simulink model "r2_b8a4x1kf"  (R2012b)
settings: Solver=VariableStepDiscrete  SolverMode=SingleTasking  StartTime=0.0  StopTime=1  RelTol=1e-3
undefined symbols (not defined in the file): fft_stages, n_bits_ants, n_bits_xengs
libraries: xbsIndex_r4 x22142, casper_library_misc x166, xbsReplacements_r4 x24, casper_library_delays x8, xps_library x5, casper_library_communications x4
(part 6 of 178)

== system r2_b8a4x1kf/bf1_ip ==
  io_delay : xbsIndex_r4/Delay  rst=off  infoeditControl=Selection of Reset will increase slice count due to use of real FFs and instead of SRLs  en=off  latency=0  dbl_ovrd=off  reg_retiming=on  block_type=delay
  r2_b8a4x1kf_new_bf1_ip_user_data_out : xbsIndex_r4/Gateway In  gui_display_data_type=Fixed-point  arith_type=Unsigned  n_bits=32  bin_pt=0  preci_type=Single  exp_width=8  frac_width=24  quantization="Round  (unbiased: +/- Inf)"  overflow=Saturate  period=1  dbl_ovrd=off  timing_constraint=None  locs_specified=off  LOCs={}  UseAsADC=off  ADCChannel='1'  inherit_from_input=off  hdl_port=on  block_type=gatewayin
  reint1 : xbsIndex_r4/Reinterpret  force_arith_type=on  arith_type=Unsigned  force_bin_pt=on  bin_pt=0  block_type=reinterpret
  sim_1 : Constant  Value=0
  slice_ip : xbsIndex_r4/Slice  nbits=32  boolean_output=off  mode=Lower Bit Location + Width  bit1=0  base1=MSB of Input  bit0=0  base0=LSB of Input  dbl_ovrd=off  block_type=slice
  in_ip : Outport
  wires:
  r2_b8a4x1kf_new_bf1_ip_user_data_out/1 -> io_delay/1
  sim_1/1 -> r2_b8a4x1kf_new_bf1_ip_user_data_out/1
  io_delay/1 -> slice_ip/1
  slice_ip/1 -> reint1/1
  reint1/1 -> in_ip/1

== system r2_b8a4x1kf/bf1_num_parts ==
  io_delay : xbsIndex_r4/Delay  rst=off  infoeditControl=Selection of Reset will increase slice count due to use of real FFs and instead of SRLs  en=off  latency=0  dbl_ovrd=off  reg_retiming=on  block_type=delay
  r2_b8a4x1kf_new_bf1_num_parts_user_data_out : xbsIndex_r4/Gateway In  gui_display_data_type=Fixed-point  arith_type=Unsigned  n_bits=32  bin_pt=0  preci_type=Single  exp_width=8  frac_width=24  quantization="Round  (unbiased: +/- Inf)"  overflow=Saturate  period=1  dbl_ovrd=off  timing_constraint=None  locs_specified=off  LOCs={}  UseAsADC=off  ADCChannel='1'  inherit_from_input=off  hdl_port=on  block_type=gatewayin
  reint1 : xbsIndex_r4/Reinterpret  force_arith_type=on  arith_type=Unsigned  force_bin_pt=on  bin_pt=0  block_type=reinterpret
  sim_1 : Constant  Value=0
  slice_n_partitions : xbsIndex_r4/Slice  nbits=6  boolean_output=off  mode=Lower Bit Location + Width  bit1=0  base1=MSB of Input  bit0=0  base0=LSB of Input  dbl_ovrd=off  block_type=slice
  in_n_partitions : Outport
  wires:
  r2_b8a4x1kf_new_bf1_num_parts_user_data_out/1 -> io_delay/1
  sim_1/1 -> r2_b8a4x1kf_new_bf1_num_parts_user_data_out/1
  io_delay/1 -> slice_n_partitions/1
  slice_n_partitions/1 -> reint1/1
  reint1/1 -> in_n_partitions/1

== system r2_b8a4x1kf/bf1_of_count ==
  out_count0 : Inport
  out_count1 : Inport  Port=2
  out_count2 : Inport  Port=3
  out_count3 : Inport  Port=4
  assert_count{0..3} (4 alike) : xbsIndex_r4/Assert  assert_type=on  type_source=Explicitly  gui_display_data_type=Fixed-point  arith_type=Unsigned  n_bits=8  bin_pt=0  preci_type=Single  exp_width=8  frac_width=24  assert_rate=off  rate_source=Explicitly  period=1  output_port=on  block_type=assert
  cast_gw : xbsIndex_r4/Convert  gui_display_data_type=Fixed-point  arith_type=Unsigned  n_bits=32  bin_pt=0  float_type=Single  exp_bits=8  fraction_bits=24  quantization=Truncate  overflow=Wrap  en=off  latency=0  dbl_ovrd=off  pipeline=off  block_type=convert
  concatenate : xbsIndex_r4/Concat  num_inputs=4  dbl_ovrd=off  block_type=concat
  io_delay : xbsIndex_r4/Delay  rst=off  infoeditControl=Selection of Reset will increase slice count due to use of real FFs and instead of SRLs  en=off  latency=0  dbl_ovrd=off  reg_retiming=on  block_type=delay
  r2_b8a4x1kf_new_bf1_of_count_user_data_in : xbsIndex_r4/Gateway Out  inherit_from_input=off  hdl_port=on  timing_constraint=None  locs_specified=off  LOCs={}  UseAsDAC=off  DACChannel='1'  block_type=gatewayout
  reint{1..4} (4 alike) : xbsIndex_r4/Reinterpret  force_arith_type=on  arith_type=Unsigned  force_bin_pt=on  bin_pt=0  block_type=reinterpret
  sim_out : Terminator
  wires:
  concatenate/1 -> io_delay/1
  io_delay/1 -> cast_gw/1
  cast_gw/1 -> r2_b8a4x1kf_new_bf1_of_count_user_data_in/1
  r2_b8a4x1kf_new_bf1_of_count_user_data_in/1 -> sim_out/1
  out_count0/1 -> assert_count0/1
  assert_count0/1 -> reint1/1
  reint1/1 -> concatenate/1
  out_count1/1 -> assert_count1/1
  assert_count1/1 -> reint2/1
  reint2/1 -> concatenate/2
  out_count2/1 -> assert_count2/1
  assert_count2/1 -> reint3/1
  reint3/1 -> concatenate/3
  out_count3/1 -> assert_count3/1
  assert_count3/1 -> reint4/1
  reint4/1 -> concatenate/4

== system r2_b8a4x1kf/bf1_out_count ==
  out_count0 : Inport
  out_count1 : Inport  Port=2
  out_count2 : Inport  Port=3
  out_count3 : Inport  Port=4
  assert_count{0..3} (4 alike) : xbsIndex_r4/Assert  assert_type=on  type_source=Explicitly  gui_display_data_type=Fixed-point  arith_type=Unsigned  n_bits=8  bin_pt=0  preci_type=Single  exp_width=8  frac_width=24  assert_rate=off  rate_source=Explicitly  period=1  output_port=on  block_type=assert
  cast_gw : xbsIndex_r4/Convert  gui_display_data_type=Fixed-point  arith_type=Unsigned  n_bits=32  bin_pt=0  float_type=Single  exp_bits=8  fraction_bits=24  quantization=Truncate  overflow=Wrap  en=off  latency=0  dbl_ovrd=off  pipeline=off  block_type=convert
  concatenate : xbsIndex_r4/Concat  num_inputs=4  dbl_ovrd=off  block_type=concat
  io_delay : xbsIndex_r4/Delay  rst=off  infoeditControl=Selection of Reset will increase slice count due to use of real FFs and instead of SRLs  en=off  latency=0  dbl_ovrd=off  reg_retiming=on  block_type=delay
  r2_b8a4x1kf_new_bf1_out_count_user_data_in : xbsIndex_r4/Gateway Out  inherit_from_input=off  hdl_port=on  timing_constraint=None  locs_specified=off  LOCs={}  UseAsDAC=off  DACChannel='1'  block_type=gatewayout
  reint{1..4} (4 alike) : xbsIndex_r4/Reinterpret  force_arith_type=on  arith_type=Unsigned  force_bin_pt=on  bin_pt=0  block_type=reinterpret
  sim_out : Terminator
  wires:
  concatenate/1 -> io_delay/1
  io_delay/1 -> cast_gw/1
  cast_gw/1 -> r2_b8a4x1kf_new_bf1_out_count_user_data_in/1
  r2_b8a4x1kf_new_bf1_out_count_user_data_in/1 -> sim_out/1
  out_count0/1 -> assert_count0/1
  assert_count0/1 -> reint1/1
  reint1/1 -> concatenate/1
  out_count1/1 -> assert_count1/1
  assert_count1/1 -> reint2/1
  reint2/1 -> concatenate/2
  out_count2/1 -> assert_count2/1
  assert_count2/1 -> reint3/1
  reint3/1 -> concatenate/3
  out_count3/1 -> assert_count3/1
  assert_count3/1 -> reint4/1
  reint4/1 -> concatenate/4

== system r2_b8a4x1kf/bf1_partitions ==
  convert1_{1..4} (4 alike) : DataTypeConversion  OutDataTypeStr=fixdt('ufix5_En0')  LockScale=on
  convert2_{1..4} (4 alike) : DataTypeConversion  OutDataTypeStr=fixdt('ufix5_En0')  ConvertRealWorld=Stored Integer (SI)  LockScale=on
  gain_1 : Gain  Gain=32768
  gain_2 : Gain  Gain=1024
  gain_3 : Gain  Gain=32
  gain_4 : Gain
  io_delay : xbsIndex_r4/Delay  rst=off  infoeditControl=Selection of Reset will increase slice count due to use of real FFs and instead of SRLs  en=off  latency=0  dbl_ovrd=off  reg_retiming=on  block_type=delay
  r2_b8a4x1kf_new_bf1_partitions_user_data_out : xbsIndex_r4/Gateway In  gui_display_data_type=Fixed-point  arith_type=Unsigned  n_bits=32  bin_pt=0  preci_type=Single  exp_width=8  frac_width=24  quantization="Round  (unbiased: +/- Inf)"  overflow=Saturate  period=1  dbl_ovrd=off  timing_constraint=None  locs_specified=off  LOCs={}  UseAsADC=off  ADCChannel='1'  inherit_from_input=off  hdl_port=on  block_type=gatewayin
  reint{1..4} (4 alike) : xbsIndex_r4/Reinterpret  force_arith_type=on  arith_type=Unsigned  force_bin_pt=on  bin_pt=0  block_type=reinterpret
  sim_{1..4} (4 alike) : Constant  Value=0
  sim_add : Sum  Inputs=++++  OutDataTypeStr=uint32
  slice_partition0_offset : xbsIndex_r4/Slice  nbits=5  boolean_output=off  mode=Lower Bit Location + Width  bit1=0  base1=MSB of Input  bit0=15  base0=LSB of Input  dbl_ovrd=off  block_type=slice
  slice_partition1_offset : xbsIndex_r4/Slice  nbits=5  boolean_output=off  mode=Lower Bit Location + Width  bit1=0  base1=MSB of Input  bit0=10  base0=LSB of Input  dbl_ovrd=off  block_type=slice
  slice_partition2_offset : xbsIndex_r4/Slice  nbits=5  boolean_output=off  mode=Lower Bit Location + Width  bit1=0  base1=MSB of Input  bit0=5  base0=LSB of Input  dbl_ovrd=off  block_type=slice
  slice_partition3_offset : xbsIndex_r4/Slice  nbits=5  boolean_output=off  mode=Lower Bit Location + Width  bit1=0  base1=MSB of Input  bit0=0  base0=LSB of Input  dbl_ovrd=off  block_type=slice
  in_partition0_offset : Outport
  in_partition1_offset : Outport  Port=2
  in_partition2_offset : Outport  Port=3
  in_partition3_offset : Outport  Port=4
  wires:
  r2_b8a4x1kf_new_bf1_partitions_user_data_out/1 -> io_delay/1
  sim_add/1 -> r2_b8a4x1kf_new_bf1_partitions_user_data_out/1
  sim_1/1 -> convert1_1/1
  convert1_1/1 -> convert2_1/1
  convert2_1/1 -> gain_1/1
  gain_1/1 -> sim_add/1
  io_delay/1 -> slice_partition0_offset/1, slice_partition1_offset/1, slice_partition2_offset/1, slice_partition3_offset/1
  slice_partition0_offset/1 -> reint1/1
  reint1/1 -> in_partition0_offset/1
  sim_2/1 -> convert1_2/1
  convert1_2/1 -> convert2_2/1
  convert2_2/1 -> gain_2/1
  gain_2/1 -> sim_add/2
  slice_partition1_offset/1 -> reint2/1
  reint2/1 -> in_partition1_offset/1
  sim_3/1 -> convert1_3/1
  convert1_3/1 -> convert2_3/1
  convert2_3/1 -> gain_3/1
  gain_3/1 -> sim_add/3
  slice_partition2_offset/1 -> reint3/1
  reint3/1 -> in_partition2_offset/1
  sim_4/1 -> convert1_4/1
  convert1_4/1 -> convert2_4/1
  convert2_4/1 -> gain_4/1
  gain_4/1 -> sim_add/4
  slice_partition3_offset/1 -> reint4/1
  reint4/1 -> in_partition3_offset/1

== system r2_b8a4x1kf/bf_config ==
  convert1_1 : DataTypeConversion  OutDataTypeStr=fixdt('ufix8_En0')  LockScale=on
  convert1_2 : DataTypeConversion  OutDataTypeStr=fixdt('ufix16_En0')  LockScale=on
  convert1_3 : DataTypeConversion  OutDataTypeStr=fixdt('ufix1_En0')  LockScale=on
  convert1_4 : DataTypeConversion  OutDataTypeStr=fixdt('ufix1_En0')  LockScale=on
  convert1_5 : DataTypeConversion  OutDataTypeStr=fixdt('ufix1_En0')  LockScale=on
  convert2_1 : DataTypeConversion  OutDataTypeStr=fixdt('ufix8_En0')  ConvertRealWorld=Stored Integer (SI)  LockScale=on
  convert2_2 : DataTypeConversion  OutDataTypeStr=fixdt('ufix16_En0')  ConvertRealWorld=Stored Integer (SI)  LockScale=on
  convert2_3 : DataTypeConversion  OutDataTypeStr=fixdt('ufix1_En0')  ConvertRealWorld=Stored Integer (SI)  LockScale=on
  convert2_4 : DataTypeConversion  OutDataTypeStr=fixdt('ufix1_En0')  ConvertRealWorld=Stored Integer (SI)  LockScale=on
  convert2_5 : DataTypeConversion  OutDataTypeStr=fixdt('ufix1_En0')  ConvertRealWorld=Stored Integer (SI)  LockScale=on
  gain_1 : Gain  Gain=524288
  gain_2 : Gain  Gain=8
  gain_3 : Gain  Gain=4
  gain_4 : Gain  Gain=2
  gain_5 : Gain
  io_delay : xbsIndex_r4/Delay  rst=off  infoeditControl=Selection of Reset will increase slice count due to use of real FFs and instead of SRLs  en=off  latency=0  dbl_ovrd=off  reg_retiming=on  block_type=delay
  r2_b8a4x1kf_new_bf_config_user_data_out : xbsIndex_r4/Gateway In  gui_display_data_type=Fixed-point  arith_type=Unsigned  n_bits=32  bin_pt=0  preci_type=Single  exp_width=8  frac_width=24  quantization="Round  (unbiased: +/- Inf)"  overflow=Saturate  period=1  dbl_ovrd=off  timing_constraint=None  locs_specified=off  LOCs={}  UseAsADC=off  ADCChannel='1'  inherit_from_input=off  hdl_port=on  block_type=gatewayin
  reint1 : xbsIndex_r4/Reinterpret  force_arith_type=on  arith_type=Unsigned  force_bin_pt=on  bin_pt=0  block_type=reinterpret
  reint2 : xbsIndex_r4/Reinterpret  force_arith_type=on  arith_type=Unsigned  force_bin_pt=on  bin_pt=0  block_type=reinterpret
  sim_{1..5} (5 alike) : Constant  Value=0
  sim_add : Sum  Inputs=+++++  OutDataTypeStr=uint32
  slice_data_id : xbsIndex_r4/Slice  nbits=8  boolean_output=off  mode=Lower Bit Location + Width  bit1=0  base1=MSB of Input  bit0=19  base0=LSB of Input  dbl_ovrd=off  block_type=slice
  slice_snap_arm : xbsIndex_r4/Slice  nbits=1  boolean_output=on  mode=Lower Bit Location + Width  bit1=0  base1=MSB of Input  bit0=1  base0=LSB of Input  dbl_ovrd=off  block_type=slice
  slice_snap_trig : xbsIndex_r4/Slice  nbits=1  boolean_output=on  mode=Lower Bit Location + Width  bit1=0  base1=MSB of Input  bit0=0  base0=LSB of Input  dbl_ovrd=off  block_type=slice
  slice_time_id : xbsIndex_r4/Slice  nbits=16  boolean_output=off  mode=Lower Bit Location + Width  bit1=0  base1=MSB of Input  bit0=3  base0=LSB of Input  dbl_ovrd=off  block_type=slice
  slice_tvg_sel : xbsIndex_r4/Slice  nbits=1  boolean_output=on  mode=Lower Bit Location + Width  bit1=0  base1=MSB of Input  bit0=2  base0=LSB of Input  dbl_ovrd=off  block_type=slice
  in_data_id : Outport
  in_time_id : Outport  Port=2
  in_tvg_sel : Outport  Port=3
  in_snap_arm : Outport  Port=4
  in_snap_trig : Outport  Port=5
  wires:
  r2_b8a4x1kf_new_bf_config_user_data_out/1 -> io_delay/1
  sim_add/1 -> r2_b8a4x1kf_new_bf_config_user_data_out/1
  sim_1/1 -> convert1_1/1
  convert1_1/1 -> convert2_1/1
  convert2_1/1 -> gain_1/1
  gain_1/1 -> sim_add/1
  io_delay/1 -> slice_data_id/1, slice_time_id/1, slice_tvg_sel/1, slice_snap_arm/1, slice_snap_trig/1
  slice_data_id/1 -> reint1/1
  reint1/1 -> in_data_id/1
  sim_2/1 -> convert1_2/1
  convert1_2/1 -> convert2_2/1
  convert2_2/1 -> gain_2/1
  gain_2/1 -> sim_add/2
  slice_time_id/1 -> reint2/1
  reint2/1 -> in_time_id/1
  sim_3/1 -> convert1_3/1
  convert1_3/1 -> convert2_3/1
  convert2_3/1 -> gain_3/1
  gain_3/1 -> sim_add/3
  slice_tvg_sel/1 -> in_tvg_sel/1
  sim_4/1 -> convert1_4/1
  convert1_4/1 -> convert2_4/1
  convert2_4/1 -> gain_4/1
  gain_4/1 -> sim_add/4
  slice_snap_arm/1 -> in_snap_arm/1
  sim_5/1 -> convert1_5/1
  convert1_5/1 -> convert2_5/1
  convert2_5/1 -> gain_5/1
  gain_5/1 -> sim_add/5
  slice_snap_trig/1 -> in_snap_trig/1

== system r2_b8a4x1kf/bf_control ==
  convert1_1 : DataTypeConversion  OutDataTypeStr=fixdt('ufix2_En0')  LockScale=on
  convert1_2 : DataTypeConversion  OutDataTypeStr=fixdt('ufix1_En0')  LockScale=on
  convert1_3 : DataTypeConversion  OutDataTypeStr=fixdt('ufix3_En0')  LockScale=on
  convert2_1 : DataTypeConversion  OutDataTypeStr=fixdt('ufix2_En0')  ConvertRealWorld=Stored Integer (SI)  LockScale=on
  convert2_2 : DataTypeConversion  OutDataTypeStr=fixdt('ufix1_En0')  ConvertRealWorld=Stored Integer (SI)  LockScale=on
  convert2_3 : DataTypeConversion  OutDataTypeStr=fixdt('ufix3_En0')  ConvertRealWorld=Stored Integer (SI)  LockScale=on
  gain_1 : Gain  Gain=16
  gain_2 : Gain  Gain=8
  gain_3 : Gain
  io_delay : xbsIndex_r4/Delay  rst=off  infoeditControl=Selection of Reset will increase slice count due to use of real FFs and instead of SRLs  en=off  latency=0  dbl_ovrd=off  reg_retiming=on  block_type=delay
  r2_b8a4x1kf_new_bf_control_user_data_out : xbsIndex_r4/Gateway In  gui_display_data_type=Fixed-point  arith_type=Unsigned  n_bits=32  bin_pt=0  preci_type=Single  exp_width=8  frac_width=24  quantization="Round  (unbiased: +/- Inf)"  overflow=Saturate  period=1  dbl_ovrd=off  timing_constraint=None  locs_specified=off  LOCs={}  UseAsADC=off  ADCChannel='1'  inherit_from_input=off  hdl_port=on  block_type=gatewayin
  reint1 : xbsIndex_r4/Reinterpret  force_arith_type=on  arith_type=Unsigned  force_bin_pt=on  bin_pt=0  block_type=reinterpret
  reint2 : xbsIndex_r4/Reinterpret  force_arith_type=on  arith_type=Unsigned  force_bin_pt=on  bin_pt=0  block_type=reinterpret
  reint3 : xbsIndex_r4/Reinterpret  force_arith_type=on  arith_type=Unsigned  force_bin_pt=on  bin_pt=0  block_type=reinterpret
  sim_1 : Constant  Value=0
  sim_2 : Constant  Value=0
  sim_3 : Constant  Value=0
  sim_add : Sum  Inputs=+++  OutDataTypeStr=uint32
  slice_antenna : xbsIndex_r4/Slice  nbits=3  boolean_output=off  mode=Lower Bit Location + Width  bit1=0  base1=MSB of Input  bit0=0  base0=LSB of Input  dbl_ovrd=off  block_type=slice
  slice_beng : xbsIndex_r4/Slice  nbits=2  boolean_output=off  mode=Lower Bit Location + Width  bit1=0  base1=MSB of Input  bit0=4  base0=LSB of Input  dbl_ovrd=off  block_type=slice
  slice_stream : xbsIndex_r4/Slice  nbits=1  boolean_output=off  mode=Lower Bit Location + Width  bit1=0  base1=MSB of Input  bit0=3  base0=LSB of Input  dbl_ovrd=off  block_type=slice
  in_beng : Outport
  in_stream : Outport  Port=2
  in_antenna : Outport  Port=3
  wires:
  r2_b8a4x1kf_new_bf_control_user_data_out/1 -> io_delay/1
  sim_add/1 -> r2_b8a4x1kf_new_bf_control_user_data_out/1
  sim_1/1 -> convert1_1/1
  convert1_1/1 -> convert2_1/1
  convert2_1/1 -> gain_1/1
  gain_1/1 -> sim_add/1
  io_delay/1 -> slice_beng/1, slice_stream/1, slice_antenna/1
  slice_beng/1 -> reint1/1
  reint1/1 -> in_beng/1
  sim_2/1 -> convert1_2/1
  convert1_2/1 -> convert2_2/1
  convert2_2/1 -> gain_2/1
  gain_2/1 -> sim_add/2
  slice_stream/1 -> reint2/1
  reint2/1 -> in_stream/1
  sim_3/1 -> convert1_3/1
  convert1_3/1 -> convert2_3/1
  convert2_3/1 -> gain_3/1
  gain_3/1 -> sim_add/3
  slice_antenna/1 -> reint3/1
  reint3/1 -> in_antenna/1

== system r2_b8a4x1kf/bf_valout_bw0 ==
  out_bw0 : Inport
  out_bw1 : Inport  Port=2
  assert_bw0 : xbsIndex_r4/Assert  assert_type=on  type_source=Explicitly  gui_display_data_type=Fixed-point  arith_type="Signed  (2's comp)"  n_bits=16  bin_pt=9  preci_type=Single  exp_width=8  frac_width=24  assert_rate=off  rate_source=Explicitly  period=1  output_port=on  block_type=assert
  assert_bw1 : xbsIndex_r4/Assert  assert_type=on  type_source=Explicitly  gui_display_data_type=Fixed-point  arith_type="Signed  (2's comp)"  n_bits=16  bin_pt=9  preci_type=Single  exp_width=8  frac_width=24  assert_rate=off  rate_source=Explicitly  period=1  output_port=on  block_type=assert
  cast_gw : xbsIndex_r4/Convert  gui_display_data_type=Fixed-point  arith_type=Unsigned  n_bits=32  bin_pt=0  float_type=Single  exp_bits=8  fraction_bits=24  quantization=Truncate  overflow=Wrap  en=off  latency=0  dbl_ovrd=off  pipeline=off  block_type=convert
  concatenate : xbsIndex_r4/Concat  num_inputs=2  dbl_ovrd=off  block_type=concat
  io_delay : xbsIndex_r4/Delay  rst=off  infoeditControl=Selection of Reset will increase slice count due to use of real FFs and instead of SRLs  en=off  latency=1  dbl_ovrd=off  reg_retiming=on  block_type=delay
  r2_b8a4x1kf_new_bf_valout_bw0_user_data_in : xbsIndex_r4/Gateway Out  inherit_from_input=off  hdl_port=on  timing_constraint=None  locs_specified=off  LOCs={}  UseAsDAC=off  DACChannel='1'  block_type=gatewayout
  reint1 : xbsIndex_r4/Reinterpret  force_arith_type=on  arith_type=Unsigned  force_bin_pt=on  bin_pt=0  block_type=reinterpret
  reint2 : xbsIndex_r4/Reinterpret  force_arith_type=on  arith_type=Unsigned  force_bin_pt=on  bin_pt=0  block_type=reinterpret
  sim_out : Terminator
  wires:
  concatenate/1 -> io_delay/1
  io_delay/1 -> cast_gw/1
  cast_gw/1 -> r2_b8a4x1kf_new_bf_valout_bw0_user_data_in/1
  r2_b8a4x1kf_new_bf_valout_bw0_user_data_in/1 -> sim_out/1
  out_bw0/1 -> assert_bw0/1
  assert_bw0/1 -> reint1/1
  reint1/1 -> concatenate/1
  out_bw1/1 -> assert_bw1/1
  assert_bw1/1 -> reint2/1
  reint2/1 -> concatenate/2

== system r2_b8a4x1kf/bf_valout_bw1 ==
  out_bw2 : Inport
  out_bw3 : Inport  Port=2
  assert_bw2 : xbsIndex_r4/Assert  assert_type=on  type_source=Explicitly  gui_display_data_type=Fixed-point  arith_type="Signed  (2's comp)"  n_bits=16  bin_pt=9  preci_type=Single  exp_width=8  frac_width=24  assert_rate=off  rate_source=Explicitly  period=1  output_port=on  block_type=assert
  assert_bw3 : xbsIndex_r4/Assert  assert_type=on  type_source=Explicitly  gui_display_data_type=Fixed-point  arith_type="Signed  (2's comp)"  n_bits=16  bin_pt=9  preci_type=Single  exp_width=8  frac_width=24  assert_rate=off  rate_source=Explicitly  period=1  output_port=on  block_type=assert
  cast_gw : xbsIndex_r4/Convert  gui_display_data_type=Fixed-point  arith_type=Unsigned  n_bits=32  bin_pt=0  float_type=Single  exp_bits=8  fraction_bits=24  quantization=Truncate  overflow=Wrap  en=off  latency=0  dbl_ovrd=off  pipeline=off  block_type=convert
  concatenate : xbsIndex_r4/Concat  num_inputs=2  dbl_ovrd=off  block_type=concat
  io_delay : xbsIndex_r4/Delay  rst=off  infoeditControl=Selection of Reset will increase slice count due to use of real FFs and instead of SRLs  en=off  latency=1  dbl_ovrd=off  reg_retiming=on  block_type=delay
  r2_b8a4x1kf_new_bf_valout_bw1_user_data_in : xbsIndex_r4/Gateway Out  inherit_from_input=off  hdl_port=on  timing_constraint=None  locs_specified=off  LOCs={}  UseAsDAC=off  DACChannel='1'  block_type=gatewayout
  reint1 : xbsIndex_r4/Reinterpret  force_arith_type=on  arith_type=Unsigned  force_bin_pt=on  bin_pt=0  block_type=reinterpret
  reint2 : xbsIndex_r4/Reinterpret  force_arith_type=on  arith_type=Unsigned  force_bin_pt=on  bin_pt=0  block_type=reinterpret
  sim_out : Terminator
  wires:
  concatenate/1 -> io_delay/1
  io_delay/1 -> cast_gw/1
  cast_gw/1 -> r2_b8a4x1kf_new_bf_valout_bw1_user_data_in/1
  r2_b8a4x1kf_new_bf_valout_bw1_user_data_in/1 -> sim_out/1
  out_bw2/1 -> assert_bw2/1
  assert_bw2/1 -> reint1/1
  reint1/1 -> concatenate/1
  out_bw3/1 -> assert_bw3/1
  assert_bw3/1 -> reint2/1
  reint2/1 -> concatenate/2

== system r2_b8a4x1kf/bf_valout_filt ==
  out_filt0 : Inport
  out_filt1 : Inport  Port=2
  out_filt2 : Inport  Port=3
  out_filt3 : Inport  Port=4
  assert_filt{0..3} (4 alike) : xbsIndex_r4/Assert  assert_type=on  type_source=Explicitly  gui_display_data_type=Fixed-point  arith_type=Unsigned  n_bits=1  bin_pt=0  preci_type=Single  exp_width=8  frac_width=24  assert_rate=off  rate_source=Explicitly  period=1  output_port=on  block_type=assert
  cast_gw : xbsIndex_r4/Convert  gui_display_data_type=Fixed-point  arith_type=Unsigned  n_bits=32  bin_pt=0  float_type=Single  exp_bits=8  fraction_bits=24  quantization=Truncate  overflow=Wrap  en=off  latency=0  dbl_ovrd=off  pipeline=off  block_type=convert
  concatenate : xbsIndex_r4/Concat  num_inputs=4  dbl_ovrd=off  block_type=concat
  io_delay : xbsIndex_r4/Delay  rst=off  infoeditControl=Selection of Reset will increase slice count due to use of real FFs and instead of SRLs  en=off  latency=1  dbl_ovrd=off  reg_retiming=on  block_type=delay
  r2_b8a4x1kf_new_bf_valout_filt_user_data_in : xbsIndex_r4/Gateway Out  inherit_from_input=off  hdl_port=on  timing_constraint=None  locs_specified=off  LOCs={}  UseAsDAC=off  DACChannel='1'  block_type=gatewayout
  reint{1..4} (4 alike) : xbsIndex_r4/Reinterpret  force_arith_type=on  arith_type=Unsigned  force_bin_pt=on  bin_pt=0  block_type=reinterpret
  sim_out : Terminator
  wires:
  concatenate/1 -> io_delay/1
  io_delay/1 -> cast_gw/1
  cast_gw/1 -> r2_b8a4x1kf_new_bf_valout_filt_user_data_in/1
  r2_b8a4x1kf_new_bf_valout_filt_user_data_in/1 -> sim_out/1
  out_filt0/1 -> assert_filt0/1
  assert_filt0/1 -> reint1/1
  reint1/1 -> concatenate/1
  out_filt1/1 -> assert_filt1/1
  assert_filt1/1 -> reint2/1
  reint2/1 -> concatenate/2
  out_filt2/1 -> assert_filt2/1
  assert_filt2/1 -> reint3/1
  reint3/1 -> concatenate/3
  out_filt3/1 -> assert_filt3/1
  assert_filt3/1 -> reint4/1
  reint4/1 -> concatenate/4

== system r2_b8a4x1kf/bf_valout_quant0 ==
  out_quant0 : Inport
  out_quant1 : Inport  Port=2
  assert_quant0 : xbsIndex_r4/Assert  assert_type=on  type_source=Explicitly  gui_display_data_type=Fixed-point  arith_type="Signed  (2's comp)"  n_bits=16  bin_pt=8  preci_type=Single  exp_width=8  frac_width=24  assert_rate=off  rate_source=Explicitly  period=1  output_port=on  block_type=assert
  assert_quant1 : xbsIndex_r4/Assert  assert_type=on  type_source=Explicitly  gui_display_data_type=Fixed-point  arith_type="Signed  (2's comp)"  n_bits=16  bin_pt=8  preci_type=Single  exp_width=8  frac_width=24  assert_rate=off  rate_source=Explicitly  period=1  output_port=on  block_type=assert
  cast_gw : xbsIndex_r4/Convert  gui_display_data_type=Fixed-point  arith_type=Unsigned  n_bits=32  bin_pt=0  float_type=Single  exp_bits=8  fraction_bits=24  quantization=Truncate  overflow=Wrap  en=off  latency=0  dbl_ovrd=off  pipeline=off  block_type=convert
  concatenate : xbsIndex_r4/Concat  num_inputs=2  dbl_ovrd=off  block_type=concat
  io_delay : xbsIndex_r4/Delay  rst=off  infoeditControl=Selection of Reset will increase slice count due to use of real FFs and instead of SRLs  en=off  latency=1  dbl_ovrd=off  reg_retiming=on  block_type=delay
  r2_b8a4x1kf_new_bf_valout_quant0_user_data_in : xbsIndex_r4/Gateway Out  inherit_from_input=off  hdl_port=on  timing_constraint=None  locs_specified=off  LOCs={}  UseAsDAC=off  DACChannel='1'  block_type=gatewayout
  reint1 : xbsIndex_r4/Reinterpret  force_arith_type=on  arith_type=Unsigned  force_bin_pt=on  bin_pt=0  block_type=reinterpret
  reint2 : xbsIndex_r4/Reinterpret  force_arith_type=on  arith_type=Unsigned  force_bin_pt=on  bin_pt=0  block_type=reinterpret
  sim_out : Terminator
  wires:
  concatenate/1 -> io_delay/1
  io_delay/1 -> cast_gw/1
  cast_gw/1 -> r2_b8a4x1kf_new_bf_valout_quant0_user_data_in/1
  r2_b8a4x1kf_new_bf_valout_quant0_user_data_in/1 -> sim_out/1
  out_quant0/1 -> assert_quant0/1
  assert_quant0/1 -> reint1/1
  reint1/1 -> concatenate/1
  out_quant1/1 -> assert_quant1/1
  assert_quant1/1 -> reint2/1
  reint2/1 -> concatenate/2

== system r2_b8a4x1kf/bf_valout_quant1 ==
  out_quant2 : Inport
  out_quant3 : Inport  Port=2
  assert_quant2 : xbsIndex_r4/Assert  assert_type=on  type_source=Explicitly  gui_display_data_type=Fixed-point  arith_type="Signed  (2's comp)"  n_bits=16  bin_pt=8  preci_type=Single  exp_width=8  frac_width=24  assert_rate=off  rate_source=Explicitly  period=1  output_port=on  block_type=assert
  assert_quant3 : xbsIndex_r4/Assert  assert_type=on  type_source=Explicitly  gui_display_data_type=Fixed-point  arith_type="Signed  (2's comp)"  n_bits=16  bin_pt=8  preci_type=Single  exp_width=8  frac_width=24  assert_rate=off  rate_source=Explicitly  period=1  output_port=on  block_type=assert
  cast_gw : xbsIndex_r4/Convert  gui_display_data_type=Fixed-point  arith_type=Unsigned  n_bits=32  bin_pt=0  float_type=Single  exp_bits=8  fraction_bits=24  quantization=Truncate  overflow=Wrap  en=off  latency=0  dbl_ovrd=off  pipeline=off  block_type=convert
  concatenate : xbsIndex_r4/Concat  num_inputs=2  dbl_ovrd=off  block_type=concat
  io_delay : xbsIndex_r4/Delay  rst=off  infoeditControl=Selection of Reset will increase slice count due to use of real FFs and instead of SRLs  en=off  latency=1  dbl_ovrd=off  reg_retiming=on  block_type=delay
  r2_b8a4x1kf_new_bf_valout_quant1_user_data_in : xbsIndex_r4/Gateway Out  inherit_from_input=off  hdl_port=on  timing_constraint=None  locs_specified=off  LOCs={}  UseAsDAC=off  DACChannel='1'  block_type=gatewayout
  reint1 : xbsIndex_r4/Reinterpret  force_arith_type=on  arith_type=Unsigned  force_bin_pt=on  bin_pt=0  block_type=reinterpret
  reint2 : xbsIndex_r4/Reinterpret  force_arith_type=on  arith_type=Unsigned  force_bin_pt=on  bin_pt=0  block_type=reinterpret
  sim_out : Terminator
  wires:
  concatenate/1 -> io_delay/1
  io_delay/1 -> cast_gw/1
  cast_gw/1 -> r2_b8a4x1kf_new_bf_valout_quant1_user_data_in/1
  r2_b8a4x1kf_new_bf_valout_quant1_user_data_in/1 -> sim_out/1
  out_quant2/1 -> assert_quant2/1
  assert_quant2/1 -> reint1/1
  reint1/1 -> concatenate/1
  out_quant3/1 -> assert_quant3/1
  assert_quant3/1 -> reint2/1
  reint2/1 -> concatenate/2

== system r2_b8a4x1kf/bf_value_ctrl ==
  convert1_{1..4} (4 alike) : DataTypeConversion  OutDataTypeStr=fixdt('ufix1_En0')  LockScale=on
  convert2_{1..4} (4 alike) : DataTypeConversion  OutDataTypeStr=fixdt('ufix1_En0')  ConvertRealWorld=Stored Integer (SI)  LockScale=on
  gain_1 : Gain  Gain=8
  gain_2 : Gain  Gain=4
  gain_3 : Gain  Gain=2
  gain_4 : Gain
  io_delay : xbsIndex_r4/Delay  rst=off  infoeditControl=Selection of Reset will increase slice count due to use of real FFs and instead of SRLs  en=off  latency=0  dbl_ovrd=off  reg_retiming=on  block_type=delay
  r2_b8a4x1kf_new_bf_value_ctrl_user_data_out : xbsIndex_r4/Gateway In  gui_display_data_type=Fixed-point  arith_type=Unsigned  n_bits=32  bin_pt=0  preci_type=Single  exp_width=8  frac_width=24  quantization="Round  (unbiased: +/- Inf)"  overflow=Saturate  period=1  dbl_ovrd=off  timing_constraint=None  locs_specified=off  LOCs={}  UseAsADC=off  ADCChannel='1'  inherit_from_input=off  hdl_port=on  block_type=gatewayin
  sim_{1..4} (4 alike) : Constant  Value=0
  sim_add : Sum  Inputs=++++  OutDataTypeStr=uint32
  slice_bw : xbsIndex_r4/Slice  nbits=1  boolean_output=on  mode=Lower Bit Location + Width  bit1=0  base1=MSB of Input  bit0=2  base0=LSB of Input  dbl_ovrd=off  block_type=slice
  slice_dupl : xbsIndex_r4/Slice  nbits=1  boolean_output=on  mode=Lower Bit Location + Width  bit1=0  base1=MSB of Input  bit0=3  base0=LSB of Input  dbl_ovrd=off  block_type=slice
  slice_filt : xbsIndex_r4/Slice  nbits=1  boolean_output=on  mode=Lower Bit Location + Width  bit1=0  base1=MSB of Input  bit0=0  base0=LSB of Input  dbl_ovrd=off  block_type=slice
  slice_quant : xbsIndex_r4/Slice  nbits=1  boolean_output=on  mode=Lower Bit Location + Width  bit1=0  base1=MSB of Input  bit0=1  base0=LSB of Input  dbl_ovrd=off  block_type=slice
  in_dupl : Outport
  in_bw : Outport  Port=2
  in_quant : Outport  Port=3
  in_filt : Outport  Port=4
  wires:
  r2_b8a4x1kf_new_bf_value_ctrl_user_data_out/1 -> io_delay/1
  sim_add/1 -> r2_b8a4x1kf_new_bf_value_ctrl_user_data_out/1
  sim_1/1 -> convert1_1/1
  convert1_1/1 -> convert2_1/1
  convert2_1/1 -> gain_1/1
  gain_1/1 -> sim_add/1
  io_delay/1 -> slice_dupl/1, slice_bw/1, slice_quant/1, slice_filt/1
  slice_dupl/1 -> in_dupl/1
  sim_2/1 -> convert1_2/1
  convert1_2/1 -> convert2_2/1
  convert2_2/1 -> gain_2/1
  gain_2/1 -> sim_add/2
  slice_bw/1 -> in_bw/1
  sim_3/1 -> convert1_3/1
  convert1_3/1 -> convert2_3/1
  convert2_3/1 -> gain_3/1
  gain_3/1 -> sim_add/3
  slice_quant/1 -> in_quant/1
  sim_4/1 -> convert1_4/1
  convert1_4/1 -> convert2_4/1
  convert2_4/1 -> gain_4/1
  gain_4/1 -> sim_add/4
  slice_filt/1 -> in_filt/1

== system r2_b8a4x1kf/bf_value_in0 ==
  convert1_1 : DataTypeConversion  OutDataTypeStr=fixdt('ufix1_En0')  LockScale=on
  convert1_2 : DataTypeConversion  OutDataTypeStr=fixdt('ufix16_En9')  LockScale=on
  convert2_1 : DataTypeConversion  OutDataTypeStr=fixdt('ufix1_En0')  ConvertRealWorld=Stored Integer (SI)  LockScale=on
  convert2_2 : DataTypeConversion  OutDataTypeStr=fixdt('ufix16_En0')  ConvertRealWorld=Stored Integer (SI)  LockScale=on
  gain_1 : Gain  Gain=65536
  gain_2 : Gain
  io_delay : xbsIndex_r4/Delay  rst=off  infoeditControl=Selection of Reset will increase slice count due to use of real FFs and instead of SRLs  en=off  latency=0  dbl_ovrd=off  reg_retiming=on  block_type=delay
  r2_b8a4x1kf_new_bf_value_in0_user_data_out : xbsIndex_r4/Gateway In  gui_display_data_type=Fixed-point  arith_type=Unsigned  n_bits=32  bin_pt=0  preci_type=Single  exp_width=8  frac_width=24  quantization="Round  (unbiased: +/- Inf)"  overflow=Saturate  period=1  dbl_ovrd=off  timing_constraint=None  locs_specified=off  LOCs={}  UseAsADC=off  ADCChannel='1'  inherit_from_input=off  hdl_port=on  block_type=gatewayin
  reint2 : xbsIndex_r4/Reinterpret  force_arith_type=on  arith_type="Signed  (2's comp)"  force_bin_pt=on  bin_pt=9  block_type=reinterpret
  sim_1 : Constant  Value=0
  sim_2 : Constant  Value=0
  sim_add : Sum  OutDataTypeStr=uint32
  slice_bw : xbsIndex_r4/Slice  nbits=16  boolean_output=off  mode=Lower Bit Location + Width  bit1=0  base1=MSB of Input  bit0=0  base0=LSB of Input  dbl_ovrd=off  block_type=slice
  slice_dupl : xbsIndex_r4/Slice  nbits=1  boolean_output=on  mode=Lower Bit Location + Width  bit1=0  base1=MSB of Input  bit0=16  base0=LSB of Input  dbl_ovrd=off  block_type=slice
  in_dupl : Outport
  in_bw : Outport  Port=2
  wires:
  r2_b8a4x1kf_new_bf_value_in0_user_data_out/1 -> io_delay/1
  sim_add/1 -> r2_b8a4x1kf_new_bf_value_in0_user_data_out/1
  sim_1/1 -> convert1_1/1
  convert1_1/1 -> convert2_1/1
  convert2_1/1 -> gain_1/1
  gain_1/1 -> sim_add/1
  io_delay/1 -> slice_dupl/1, slice_bw/1
  slice_dupl/1 -> in_dupl/1
  sim_2/1 -> convert1_2/1
  convert1_2/1 -> convert2_2/1
  convert2_2/1 -> gain_2/1
  gain_2/1 -> sim_add/2
  slice_bw/1 -> reint2/1
  reint2/1 -> in_bw/1

== system r2_b8a4x1kf/bf_value_in1 ==
  convert1_1 : DataTypeConversion  OutDataTypeStr=fixdt('ufix16_En8')  LockScale=on
  convert1_2 : DataTypeConversion  OutDataTypeStr=fixdt('ufix1_En0')  LockScale=on
  convert2_1 : DataTypeConversion  OutDataTypeStr=fixdt('ufix16_En0')  ConvertRealWorld=Stored Integer (SI)  LockScale=on
  convert2_2 : DataTypeConversion  OutDataTypeStr=fixdt('ufix1_En0')  ConvertRealWorld=Stored Integer (SI)  LockScale=on
  gain_1 : Gain  Gain=2
  gain_2 : Gain
  io_delay : xbsIndex_r4/Delay  rst=off  infoeditControl=Selection of Reset will increase slice count due to use of real FFs and instead of SRLs  en=off  latency=0  dbl_ovrd=off  reg_retiming=on  block_type=delay
  r2_b8a4x1kf_new_bf_value_in1_user_data_out : xbsIndex_r4/Gateway In  gui_display_data_type=Fixed-point  arith_type=Unsigned  n_bits=32  bin_pt=0  preci_type=Single  exp_width=8  frac_width=24  quantization="Round  (unbiased: +/- Inf)"  overflow=Saturate  period=1  dbl_ovrd=off  timing_constraint=None  locs_specified=off  LOCs={}  UseAsADC=off  ADCChannel='1'  inherit_from_input=off  hdl_port=on  block_type=gatewayin
  reint1 : xbsIndex_r4/Reinterpret  force_arith_type=on  arith_type="Signed  (2's comp)"  force_bin_pt=on  bin_pt=8  block_type=reinterpret
  sim_1 : Constant  Value=0
  sim_2 : Constant  Value=0
  sim_add : Sum  OutDataTypeStr=uint32
  slice_filt : xbsIndex_r4/Slice  nbits=1  boolean_output=on  mode=Lower Bit Location + Width  bit1=0  base1=MSB of Input  bit0=0  base0=LSB of Input  dbl_ovrd=off  block_type=slice
  slice_quant : xbsIndex_r4/Slice  nbits=16  boolean_output=off  mode=Lower Bit Location + Width  bit1=0  base1=MSB of Input  bit0=1  base0=LSB of Input  dbl_ovrd=off  block_type=slice
  in_quant : Outport
  in_filt : Outport  Port=2
  wires:
  r2_b8a4x1kf_new_bf_value_in1_user_data_out/1 -> io_delay/1
  sim_add/1 -> r2_b8a4x1kf_new_bf_value_in1_user_data_out/1
  sim_1/1 -> convert1_1/1
  convert1_1/1 -> convert2_1/1
  convert2_1/1 -> gain_1/1
  gain_1/1 -> sim_add/1
  io_delay/1 -> slice_quant/1, slice_filt/1
  slice_quant/1 -> reint1/1
  reint1/1 -> in_quant/1
  sim_2/1 -> convert1_2/1
  convert1_2/1 -> convert2_2/1
  convert2_2/1 -> gain_2/1
  gain_2/1 -> sim_add/2
  slice_filt/1 -> in_filt/1

== system r2_b8a4x1kf/bfsnap_out ==
  in_sync : Inport
  in_en : Inport  Port=2
  in_d32 : Inport  Port=3
  in_time27 : Inport  Port=4
  we : Inport  Port=5
  trig : Inport  Port=6
  assert_d32 : xbsIndex_r4/Assert  assert_type=on  type_source=Explicitly  gui_display_data_type=Fixed-point  arith_type=Unsigned  n_bits=32  bin_pt=0  preci_type=Single  exp_width=8  frac_width=24  assert_rate=off  rate_source=Explicitly  period=1  output_port=on  block_type=assert
  assert_en : xbsIndex_r4/Assert  assert_type=on  type_source=Explicitly  gui_display_data_type=Boolean  arith_type=Boolean  n_bits=1  bin_pt=0  preci_type=Single  exp_width=8  frac_width=24  assert_rate=off  rate_source=Explicitly  period=1  output_port=on  block_type=assert
  assert_sync : xbsIndex_r4/Assert  assert_type=on  type_source=Explicitly  gui_display_data_type=Boolean  arith_type=Boolean  n_bits=1  bin_pt=0  preci_type=Single  exp_width=8  frac_width=24  assert_rate=off  rate_source=Explicitly  period=1  output_port=on  block_type=assert
  assert_time27 : xbsIndex_r4/Assert  assert_type=on  type_source=Explicitly  gui_display_data_type=Fixed-point  arith_type=Unsigned  n_bits=27  bin_pt=0  preci_type=Single  exp_width=8  frac_width=24  assert_rate=off  rate_source=Explicitly  period=1  output_port=on  block_type=assert
  buscreate : Subsystem  AncestorBlock=casper_library_flow_control/bus_create  mask(bus_create){inputNum=4}
      mask prompts: inputNum "Number of inputs:"
      mask init:
      | bus_create_init(gcb,...
      |     'inputNum', inputNum);
  ss : Subsystem  Tag=casper:snapshot  AncestorBlock=casper_library_scopes/snapshot  mask(snapshot){storage=bram, dram_dimm=2, dram_clock=250, nsamples=12, data_width=64, offset=on, circap=off, value=off, use_dsp48=on}
      mask prompts: storage "Storage medium"; dram_dimm "DRAM dimm"; dram_clock "DRAM clock rate"; nsamples "Number of Samples (2^?)"; data_width "Data width"; offset "Start delay support"; circap "Circular capture support"; value "Extra value capture support"; use_dsp48 "Use DSP48s to implement counters"
      mask help:
      | Standard snap block, but with the following optional extras;
      |  1) Optionally delay the fabric trigger by a user-specified number of valids.
      |  2) Capture continuously after a trigger until a stop pulse is received. Data is captured into BRAM continuously, with old data being overwritten until a stop command is received. Then stop capturing when memory is filled. This enables you to get some data before and some data after the stop pulse. Use the 'tr_en_cnt' register to determine where you are in your vector. 'Addr' register's MSb now indicates 'busy capturing'.
      |  3) Optionally capture a value on an input port to a register at the same time as the first data sample.
      |  4) Implement counters using DSP48Es to save resources.
      mask init:
      | snapshot_init(gcb, ...
      |     'storage', storage, ...
      |     'dram_dimm', dram_dimm, ...
      |     'dram_clock', dram_clock, ...
      |     'nsamples', nsamples, ...
      |     'data_width', data_width, ...
      |     'offset', offset, ...
      |     'circap', circap, ...
      |     'value', value, ...
      |     'use_dsp48', use_dsp48);
      mask TypeOptions storage: bram | dram
      mask Callback storage: snapshot_callback();
      mask TypeOptions dram_dimm: 1 | 2 | 3 | 4
      mask TypeOptions dram_clock: 200 | 250 | 266 | 300 | 333
      mask TypeOptions data_width: 8 | 16 | 32 | 64 | 128
  wires:
  buscreate/1(bus_out) -> ss/1(din)
  in_sync/1 -> assert_sync/1
  assert_sync/1 -> buscreate/1(in1)
  in_en/1 -> assert_en/1
  assert_en/1 -> buscreate/2(in2)
  in_d32/1 -> assert_d32/1
  assert_d32/1 -> buscreate/3(in3)
  in_time27/1 -> assert_time27/1
  assert_time27/1 -> buscreate/4(in4)
  we/1 -> ss/2(we)
  trig/1 -> ss/3(trig)

== system r2_b8a4x1kf/board_id ==
  io_delay : xbsIndex_r4/Delay  rst=off  infoeditControl=Selection of Reset will increase slice count due to use of real FFs and instead of SRLs  en=off  latency=0  dbl_ovrd=off  reg_retiming=on  block_type=delay
  r2_b8a4x1kf_new_board_id_user_data_out : xbsIndex_r4/Gateway In  gui_display_data_type=Fixed-point  arith_type=Unsigned  n_bits=32  bin_pt=0  preci_type=Single  exp_width=8  frac_width=24  quantization="Round  (unbiased: +/- Inf)"  overflow=Saturate  period=1  dbl_ovrd=off  timing_constraint=None  locs_specified=off  LOCs={}  UseAsADC=off  ADCChannel='1'  inherit_from_input=off  hdl_port=on  block_type=gatewayin
  reint1 : xbsIndex_r4/Reinterpret  force_arith_type=on  arith_type=Unsigned  force_bin_pt=on  bin_pt=0  block_type=reinterpret
  sim_1 : Constant  Value=0
  slice_reg : xbsIndex_r4/Slice  nbits=32  boolean_output=off  mode=Lower Bit Location + Width  bit1=0  base1=MSB of Input  bit0=0  base0=LSB of Input  dbl_ovrd=off  block_type=slice
  in_reg : Outport
  wires:
  r2_b8a4x1kf_new_board_id_user_data_out/1 -> io_delay/1
  sim_1/1 -> r2_b8a4x1kf_new_board_id_user_data_out/1
  io_delay/1 -> slice_reg/1
  slice_reg/1 -> reint1/1
  reint1/1 -> in_reg/1

== system r2_b8a4x1kf/bus_expand ==
  bus_in : Inport
  slice1 : xbsIndex_r4/Slice  nbits=1  boolean_output=on  mode=Upper Bit Location + Width  bit1=-5  base1=MSB of Input  bit0=0  base0=LSB of Input  dbl_ovrd=off  block_type=slice
  slice2 : xbsIndex_r4/Slice  nbits=1  boolean_output=on  mode=Upper Bit Location + Width  bit1=-4  base1=MSB of Input  bit0=0  base0=LSB of Input  dbl_ovrd=off  block_type=slice
  slice3 : xbsIndex_r4/Slice  nbits=1  boolean_output=on  mode=Upper Bit Location + Width  bit1=-3  base1=MSB of Input  bit0=0  base0=LSB of Input  dbl_ovrd=off  block_type=slice
  slice4 : xbsIndex_r4/Slice  nbits=1  boolean_output=on  mode=Upper Bit Location + Width  bit1=-2  base1=MSB of Input  bit0=0  base0=LSB of Input  dbl_ovrd=off  block_type=slice
  slice5 : xbsIndex_r4/Slice  nbits=1  boolean_output=on  mode=Upper Bit Location + Width  bit1=-1  base1=MSB of Input  bit0=0  base0=LSB of Input  dbl_ovrd=off  block_type=slice
  slice6 : xbsIndex_r4/Slice  nbits=1  boolean_output=on  mode=Upper Bit Location + Width  bit1=0  base1=MSB of Input  bit0=0  base0=LSB of Input  dbl_ovrd=off  block_type=slice
  msb_out6 : Outport
  out5 : Outport  Port=2
  out4 : Outport  Port=3
  out3 : Outport  Port=4
  out2 : Outport  Port=5
  lsb_out1 : Outport  Port=6
  wires:
  bus_in/1 -> slice6/1, slice5/1, slice4/1, slice3/1, slice2/1, slice1/1
  slice6/1 -> msb_out6/1
  slice5/1 -> out5/1
  slice4/1 -> out4/1
  slice3/1 -> out3/1
  slice2/1 -> out2/1
  slice1/1 -> lsb_out1/1

== system r2_b8a4x1kf/bus_expand1 ==
  bus_in : Inport
  slice1 : xbsIndex_r4/Slice  nbits=1  boolean_output=on  mode=Upper Bit Location + Width  bit1=-4  base1=MSB of Input  bit0=0  base0=LSB of Input  dbl_ovrd=off  block_type=slice
  slice2 : xbsIndex_r4/Slice  nbits=1  boolean_output=on  mode=Upper Bit Location + Width  bit1=-3  base1=MSB of Input  bit0=0  base0=LSB of Input  dbl_ovrd=off  block_type=slice
  slice3 : xbsIndex_r4/Slice  nbits=1  boolean_output=on  mode=Upper Bit Location + Width  bit1=-2  base1=MSB of Input  bit0=0  base0=LSB of Input  dbl_ovrd=off  block_type=slice
  slice4 : xbsIndex_r4/Slice  nbits=1  boolean_output=on  mode=Upper Bit Location + Width  bit1=-1  base1=MSB of Input  bit0=0  base0=LSB of Input  dbl_ovrd=off  block_type=slice
  slice5 : xbsIndex_r4/Slice  nbits=1  boolean_output=on  mode=Upper Bit Location + Width  bit1=0  base1=MSB of Input  bit0=0  base0=LSB of Input  dbl_ovrd=off  block_type=slice
  msb_out5 : Outport
  out4 : Outport  Port=2
  out3 : Outport  Port=3
  out2 : Outport  Port=4
  lsb_out1 : Outport  Port=5
  wires:
  slice1/1 -> lsb_out1/1
  slice2/1 -> out2/1
  slice3/1 -> out3/1
  slice4/1 -> out4/1
  slice5/1 -> msb_out5/1
  bus_in/1 -> slice1/1, slice2/1, slice3/1, slice4/1, slice5/1

== system r2_b8a4x1kf/bus_expand2 ==
  bus_in : Inport
  slice1 : xbsIndex_r4/Slice  nbits=1  boolean_output=on  mode=Upper Bit Location + Width  bit1=-4  base1=MSB of Input  bit0=0  base0=LSB of Input  dbl_ovrd=off  block_type=slice
  slice2 : xbsIndex_r4/Slice  nbits=1  boolean_output=on  mode=Upper Bit Location + Width  bit1=-3  base1=MSB of Input  bit0=0  base0=LSB of Input  dbl_ovrd=off  block_type=slice
  slice3 : xbsIndex_r4/Slice  nbits=1  boolean_output=on  mode=Upper Bit Location + Width  bit1=-2  base1=MSB of Input  bit0=0  base0=LSB of Input  dbl_ovrd=off  block_type=slice
  slice4 : xbsIndex_r4/Slice  nbits=1  boolean_output=on  mode=Upper Bit Location + Width  bit1=-1  base1=MSB of Input  bit0=0  base0=LSB of Input  dbl_ovrd=off  block_type=slice
  slice5 : xbsIndex_r4/Slice  nbits=1  boolean_output=on  mode=Upper Bit Location + Width  bit1=0  base1=MSB of Input  bit0=0  base0=LSB of Input  dbl_ovrd=off  block_type=slice
  msb_out5 : Outport
  out4 : Outport  Port=2
  out3 : Outport  Port=3
  out2 : Outport  Port=4
  lsb_out1 : Outport  Port=5
  wires:
  bus_in/1 -> slice5/1, slice4/1, slice3/1, slice2/1, slice1/1
  slice5/1 -> msb_out5/1
  slice4/1 -> out4/1
  slice3/1 -> out3/1
  slice2/1 -> out2/1
  slice1/1 -> lsb_out1/1

== system r2_b8a4x1kf/bus_expand3 ==
  bus_in : Inport
  slice1 : xbsIndex_r4/Slice  nbits=1  boolean_output=on  mode=Upper Bit Location + Width  bit1=-5  base1=MSB of Input  bit0=0  base0=LSB of Input  dbl_ovrd=off  block_type=slice
  slice2 : xbsIndex_r4/Slice  nbits=1  boolean_output=on  mode=Upper Bit Location + Width  bit1=-4  base1=MSB of Input  bit0=0  base0=LSB of Input  dbl_ovrd=off  block_type=slice
  slice3 : xbsIndex_r4/Slice  nbits=1  boolean_output=on  mode=Upper Bit Location + Width  bit1=-3  base1=MSB of Input  bit0=0  base0=LSB of Input  dbl_ovrd=off  block_type=slice
  slice4 : xbsIndex_r4/Slice  nbits=1  boolean_output=on  mode=Upper Bit Location + Width  bit1=-2  base1=MSB of Input  bit0=0  base0=LSB of Input  dbl_ovrd=off  block_type=slice
  slice5 : xbsIndex_r4/Slice  nbits=1  boolean_output=on  mode=Upper Bit Location + Width  bit1=-1  base1=MSB of Input  bit0=0  base0=LSB of Input  dbl_ovrd=off  block_type=slice
  slice6 : xbsIndex_r4/Slice  nbits=1  boolean_output=on  mode=Upper Bit Location + Width  bit1=0  base1=MSB of Input  bit0=0  base0=LSB of Input  dbl_ovrd=off  block_type=slice
  msb_out6 : Outport
  out5 : Outport  Port=2
  out4 : Outport  Port=3
  out3 : Outport  Port=4
  out2 : Outport  Port=5
  lsb_out1 : Outport  Port=6
  wires:
  slice1/1 -> lsb_out1/1
  slice2/1 -> out2/1
  slice3/1 -> out3/1
  slice4/1 -> out4/1
  slice5/1 -> out5/1
  slice6/1 -> msb_out6/1
  bus_in/1 -> slice1/1, slice2/1, slice3/1, slice4/1, slice5/1, slice6/1

== system r2_b8a4x1kf/bus_expand4 ==
  bus_in : Inport
  slice1 : xbsIndex_r4/Slice  nbits=1  boolean_output=on  mode=Upper Bit Location + Width  bit1=-4  base1=MSB of Input  bit0=0  base0=LSB of Input  dbl_ovrd=off  block_type=slice
  slice2 : xbsIndex_r4/Slice  nbits=1  boolean_output=on  mode=Upper Bit Location + Width  bit1=-3  base1=MSB of Input  bit0=0  base0=LSB of Input  dbl_ovrd=off  block_type=slice
  slice3 : xbsIndex_r4/Slice  nbits=1  boolean_output=on  mode=Upper Bit Location + Width  bit1=-2  base1=MSB of Input  bit0=0  base0=LSB of Input  dbl_ovrd=off  block_type=slice
  slice4 : xbsIndex_r4/Slice  nbits=1  boolean_output=on  mode=Upper Bit Location + Width  bit1=-1  base1=MSB of Input  bit0=0  base0=LSB of Input  dbl_ovrd=off  block_type=slice
  slice5 : xbsIndex_r4/Slice  nbits=1  boolean_output=on  mode=Upper Bit Location + Width  bit1=0  base1=MSB of Input  bit0=0  base0=LSB of Input  dbl_ovrd=off  block_type=slice
  msb_out5 : Outport
  out4 : Outport  Port=2
  out3 : Outport  Port=3
  out2 : Outport  Port=4
  lsb_out1 : Outport  Port=5
  wires:
  slice1/1 -> lsb_out1/1
  slice2/1 -> out2/1
  slice3/1 -> out3/1
  slice4/1 -> out4/1
  slice5/1 -> msb_out5/1
  bus_in/1 -> slice1/1, slice2/1, slice3/1, slice4/1, slice5/1

== system r2_b8a4x1kf/bus_expand5 ==
  bus_in : Inport
  reinterpret1 : xbsIndex_r4/Reinterpret  force_arith_type=on  arith_type=Unsigned  force_bin_pt=on  bin_pt=0  block_type=reinterpret
  reinterpret2 : xbsIndex_r4/Reinterpret  force_arith_type=on  arith_type=Unsigned  force_bin_pt=on  bin_pt=0  block_type=reinterpret
  slice1 : xbsIndex_r4/Slice  nbits=16  boolean_output=off  mode=Upper Bit Location + Width  bit1=-16  base1=MSB of Input  bit0=0  base0=LSB of Input  dbl_ovrd=off  block_type=slice
  slice2 : xbsIndex_r4/Slice  nbits=16  boolean_output=off  mode=Upper Bit Location + Width  bit1=0  base1=MSB of Input  bit0=0  base0=LSB of Input  dbl_ovrd=off  block_type=slice
  msb_out2 : Outport
  lsb_out1 : Outport  Port=2
  wires:
  bus_in/1 -> slice2/1, slice1/1
  slice2/1 -> reinterpret2/1
  reinterpret2/1 -> msb_out2/1
  slice1/1 -> reinterpret1/1
  reinterpret1/1 -> lsb_out1/1

== system r2_b8a4x1kf/bus_expand6 ==
  bus_in : Inport
  reinterpret1 : xbsIndex_r4/Reinterpret  force_arith_type=on  arith_type=Unsigned  force_bin_pt=on  bin_pt=0  block_type=reinterpret
  reinterpret2 : xbsIndex_r4/Reinterpret  force_arith_type=on  arith_type=Unsigned  force_bin_pt=on  bin_pt=0  block_type=reinterpret
  slice1 : xbsIndex_r4/Slice  nbits=16  boolean_output=off  mode=Upper Bit Location + Width  bit1=-16  base1=MSB of Input  bit0=0  base0=LSB of Input  dbl_ovrd=off  block_type=slice
  slice2 : xbsIndex_r4/Slice  nbits=16  boolean_output=off  mode=Upper Bit Location + Width  bit1=0  base1=MSB of Input  bit0=0  base0=LSB of Input  dbl_ovrd=off  block_type=slice
  msb_out2 : Outport
  lsb_out1 : Outport  Port=2
  wires:
  reinterpret1/1 -> lsb_out1/1
  slice1/1 -> reinterpret1/1
  reinterpret2/1 -> msb_out2/1
  slice2/1 -> reinterpret2/1
  bus_in/1 -> slice1/1, slice2/1

== system r2_b8a4x1kf/bus_expand7 ==
  bus_in : Inport
  reinterpret1 : xbsIndex_r4/Reinterpret  force_arith_type=on  arith_type=Unsigned  force_bin_pt=on  bin_pt=0  block_type=reinterpret
  reinterpret2 : xbsIndex_r4/Reinterpret  force_arith_type=on  arith_type=Unsigned  force_bin_pt=on  bin_pt=0  block_type=reinterpret
  slice1 : xbsIndex_r4/Slice  nbits=16  boolean_output=off  mode=Upper Bit Location + Width  bit1=-16  base1=MSB of Input  bit0=0  base0=LSB of Input  dbl_ovrd=off  block_type=slice
  slice2 : xbsIndex_r4/Slice  nbits=16  boolean_output=off  mode=Upper Bit Location + Width  bit1=0  base1=MSB of Input  bit0=0  base0=LSB of Input  dbl_ovrd=off  block_type=slice
  msb_out2 : Outport
  lsb_out1 : Outport  Port=2
  wires:
  reinterpret1/1 -> lsb_out1/1
  slice1/1 -> reinterpret1/1
  reinterpret2/1 -> msb_out2/1
  slice2/1 -> reinterpret2/1
  bus_in/1 -> slice1/1, slice2/1
